simulink model "inout_test"  (Simulink 4.00)
settings: Solver=ode45  StartTime=0.0  StopTime=10.0  RelTol=1e-3
libraries: simulink3 x1
settings Model: BlockReductionOpt=off

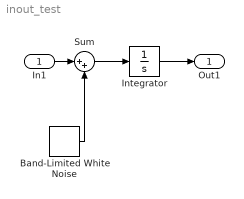
== system inout_test ==
  In1 : Inport  Port=1
  Band-Limited White Noise : simulink3/Sources/Band-Limited White Noise  Cov=[0.1]  Ts=0.1  seed=[23341]
  Integrator : Integrator  ExternalReset=none  InitialConditionSource=internal  InitialCondition=-1  LimitOutput=off  UpperSaturationLimit=inf  LowerSaturationLimit=-inf  ShowSaturationPort=off  ShowStatePort=off  AbsoluteTolerance=auto
  Sum : Sum  Inputs=|++  SaturateOnIntegerOverflow=on
  Out1 : Outport  Port=1
  wires:
  In1/1 -> Sum/1
  Integrator/1 -> Out1/1
  Band-Limited White Noise/1 -> Sum/2
  Sum/1 -> Integrator/1
